simulink model "case_09_30_to_2_to_0"  (R2025b)
settings: Solver=VariableStepAuto  StartTime=0.0  StopTime=120  RelTol=1e-3
settings Model: Creator=sanborkl  LastModifiedBy=sanborkl
settings DebuggingCC: UnderSpecifiedDimensionMsg=warning

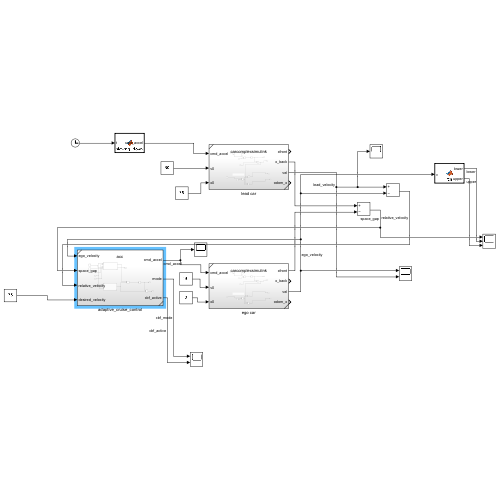
[thumbnail: Simulink's stored preview of the top-level diagram]
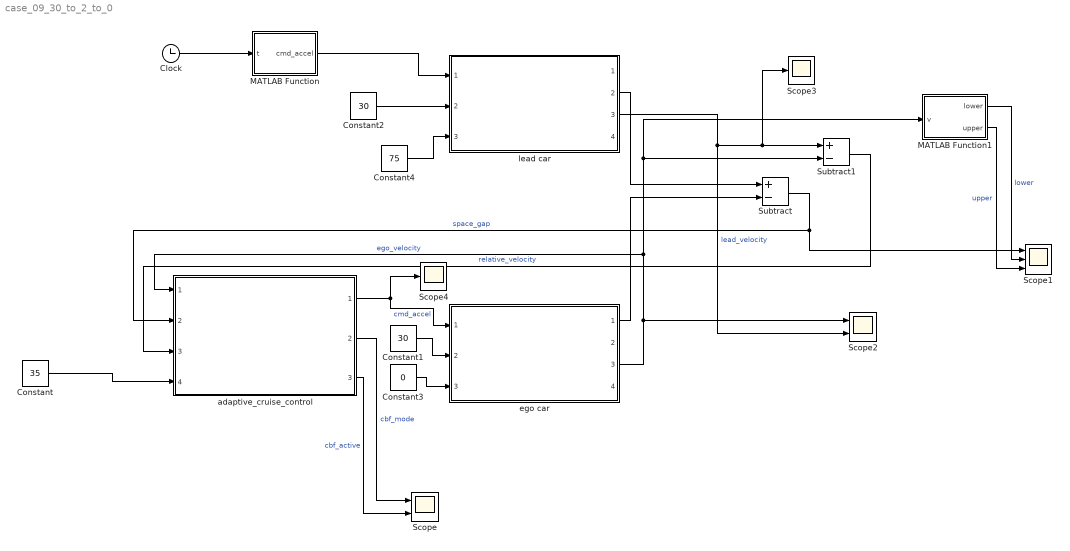
== system case_09_30_to_2_to_0 ==
  Clock : Clock
  Constant : Constant  Value=35
  Constant1 : Constant  Value=30
  Constant2 : Constant  Value=30
  Constant3 : Constant  Value=0
  Constant4 : Constant  Value=75
  MATLAB Function : MATLAB Function  TreatAsAtomicUnit=on
  MATLAB Function1 : MATLAB Function  TreatAsAtomicUnit=on
  Scope : Scope  NumInputPorts=2
      settings: ActiveDisplayYMinimum=0.875  ActiveDisplayYMaximum=2.125
  Scope1 : Scope  NumInputPorts=3
      settings: ActiveDisplayYMinimum=4.0434336146513088  ActiveDisplayYMaximum=12.021964247104087  YLabel=m
  Scope2 : Scope  NumInputPorts=2
      settings: ActiveDisplayYMinimum=-3.7499999999999991  ActiveDisplayYMaximum=33.75  YLabel=m/s  DataLoggingVariableName=ScopeData2
  Scope3 : Scope
      settings: ActiveDisplayYMinimum=-3.7499999999999991  ActiveDisplayYMaximum=33.75  YLabel=m/s  DataLoggingVariableName=ScopeData3
  Scope4 : Scope
      settings: ActiveDisplayYMinimum=-0.59172127752787473  ActiveDisplayYMaximum=0.15722343576848719  YLabel=m/s^2  DataLoggingVariableName=ScopeData7
  Subtract : Sum  Inputs=+-
  Subtract1 : Sum  Inputs=+-
  adaptive_cruise_control : Subsystem  ReferencedSubsystem=acc
  ego car : Subsystem  ReferencedSubsystem=carcomplexsimulink
  lead car : Subsystem  ReferencedSubsystem=carcomplexsimulink
  wires:
  adaptive_cruise_control/1 -> ego car/1, Scope4/1  "cmd_accel"
  ego car/3 -> MATLAB Function1/1(v), Subtract1/2, adaptive_cruise_control/1, Scope2/1  "ego_velocity"
  lead car/2 -> Subtract/1
  ego car/1 -> Subtract/2
  Subtract/1 -> Scope1/1, adaptive_cruise_control/2  "space_gap"
  lead car/3 -> Scope2/2, Scope3/1, Subtract1/1  "lead_velocity"
  Subtract1/1 -> adaptive_cruise_control/3  "relative_velocity"
  Constant/1 -> adaptive_cruise_control/4
  adaptive_cruise_control/2 -> Scope/1  "cbf_mode"
  Constant1/1 -> ego car/2
  Constant2/1 -> lead car/2
  Constant3/1 -> ego car/3
  Constant4/1 -> lead car/3
  MATLAB Function/1(cmd_accel) -> lead car/1
  adaptive_cruise_control/3 -> Scope/2  "cbf_active"
  Clock/1 -> MATLAB Function/1(t)
  MATLAB Function1/1(lower) -> Scope1/2  "lower"
  MATLAB Function1/2(upper) -> Scope1/3  "upper"

== matlab function case_09_30_to_2_to_0/MATLAB Function ==
  data: t input; cmd_accel output
function cmd_accel = slowing_down(t)

if t < 30
    cmd_accel = 0;
elseif t >= 30 && t < 58
    cmd_accel = -1;
elseif t >= 58 && t < 90
    cmd_accel = 0;
elseif t >= 90 && t < 100
    cmd_accel = -0.5;
else
    cmd_accel = 0;
end

== matlab function case_09_30_to_2_to_0/MATLAB Function1 ==
  data: v input; lower output; upper output
function [lower, upper] = fcn(v)

lower = 2 * v + 5;
upper = 2 * v + 15;
